simulink model "p2p_microgrid"  (R2024b)
settings: Solver=ode45  StartTime=0.0  StopTime=28800  MaxStep=1  MinStep=0.001  RelTol=1e-3
settings Model: Creator=user  LastModifiedBy=user
settings SolverCC: AlgebraicLoopSolver=LineSearch
settings DebuggingCC: AlgebraicLoopMsg=none

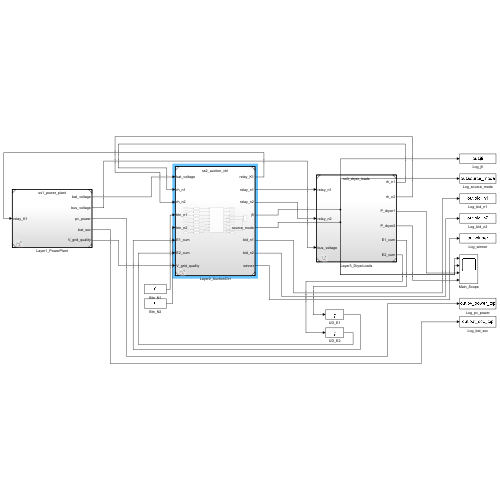
[thumbnail: Simulink's stored preview of the top-level diagram]
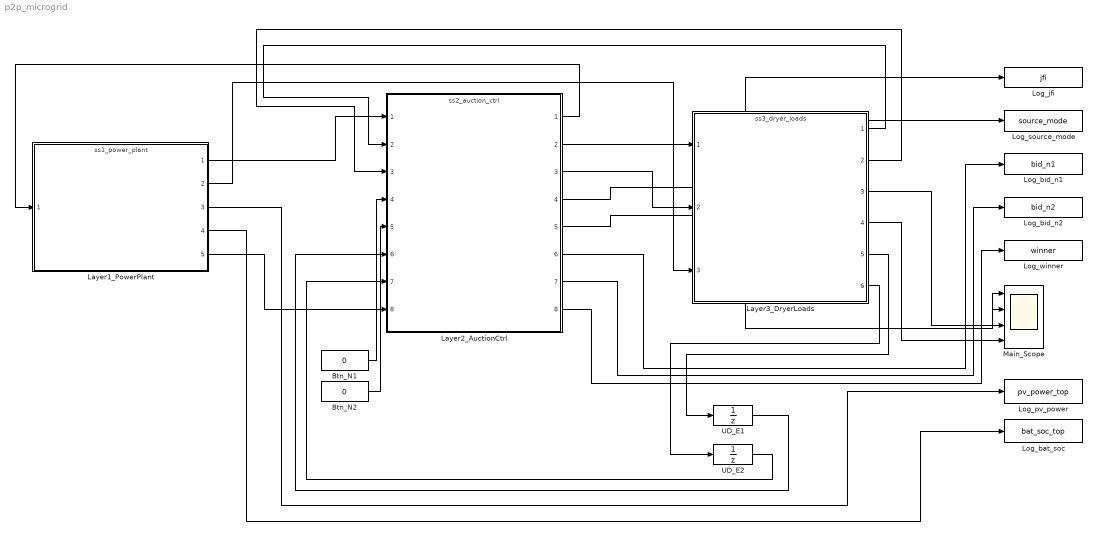
== system p2p_microgrid ==
  Btn_N1 : Constant  Value=0
  Btn_N2 : Constant  Value=0
  Layer1_PowerPlant : ModelReference  ModelNameDialog=ss1_power_plant  SimulationMode=Normal  ModelReferenceVersion=1.16
  Layer2_AuctionCtrl : ModelReference  ModelNameDialog=ss2_auction_ctrl  SimulationMode=Normal  ModelReferenceVersion=1.4
  Layer3_DryerLoads : ModelReference  ModelNameDialog=ss3_dryer_loads  SimulationMode=Normal  ModelReferenceVersion=1.2
  Log_bat_soc : ToWorkspace  VariableName=bat_soc_top  SampleTime=-1
  Log_bid_n1 : ToWorkspace  VariableName=bid_n1  SampleTime=-1
  Log_bid_n2 : ToWorkspace  VariableName=bid_n2  SampleTime=-1
  Log_jfi : ToWorkspace  VariableName=jfi  SampleTime=-1
  Log_pv_power : ToWorkspace  VariableName=pv_power_top  SampleTime=-1
  Log_source_mode : ToWorkspace  VariableName=source_mode  SampleTime=-1
  Log_winner : ToWorkspace  VariableName=winner  SampleTime=-1
  Main_Scope : Scope  NumInputPorts=4
  UD_E1 : UnitDelay  SampleTime=10  HasFrameUpgradeWarning=on
  UD_E2 : UnitDelay  SampleTime=10  HasFrameUpgradeWarning=on
  wires:
  Layer1_PowerPlant/1 -> Layer2_AuctionCtrl/1
  Layer3_DryerLoads/1 -> Layer2_AuctionCtrl/2
  Layer3_DryerLoads/2 -> Layer2_AuctionCtrl/3
  Btn_N1/1 -> Layer2_AuctionCtrl/4
  Btn_N2/1 -> Layer2_AuctionCtrl/5
  Layer2_AuctionCtrl/1 -> Layer1_PowerPlant/1
  Layer2_AuctionCtrl/2 -> Layer3_DryerLoads/1
  Layer2_AuctionCtrl/3 -> Layer3_DryerLoads/2
  Layer1_PowerPlant/2 -> Layer3_DryerLoads/3
  Layer2_AuctionCtrl/4 -> Log_jfi/1, Main_Scope/1
  Layer2_AuctionCtrl/5 -> Log_source_mode/1, Main_Scope/2
  Layer2_AuctionCtrl/6 -> Log_bid_n1/1
  Layer2_AuctionCtrl/7 -> Log_bid_n2/1
  Layer2_AuctionCtrl/8 -> Log_winner/1
  Layer3_DryerLoads/3 -> Main_Scope/3
  Layer3_DryerLoads/4 -> Main_Scope/4
  Layer3_DryerLoads/5 -> UD_E1/1
  UD_E1/1 -> Layer2_AuctionCtrl/6
  Layer3_DryerLoads/6 -> UD_E2/1
  UD_E2/1 -> Layer2_AuctionCtrl/7
  Layer1_PowerPlant/5 -> Layer2_AuctionCtrl/8
  Layer1_PowerPlant/3 -> Log_pv_power/1
  Layer1_PowerPlant/4 -> Log_bat_soc/1
